simulink model "thermostate"  (R2026a)
settings: Solver=VariableStepAuto  StopTime=1800
undefined symbols (not defined in the file): cp, eta, m_water, P_heater, T_ambient, T_high, T_initial, T_low, t_stop, UA
settings Model: Creator=a  LastModifiedBy=a

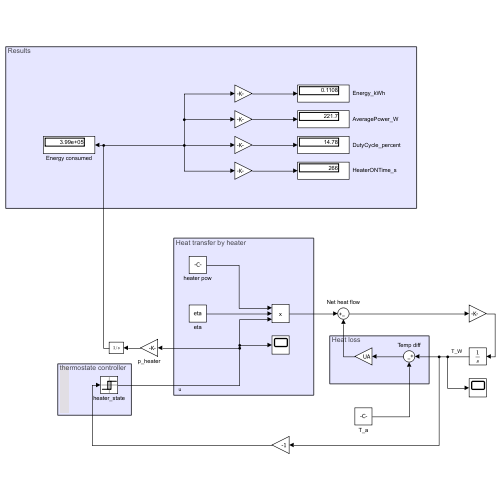
[thumbnail: Simulink's stored preview of the top-level diagram]
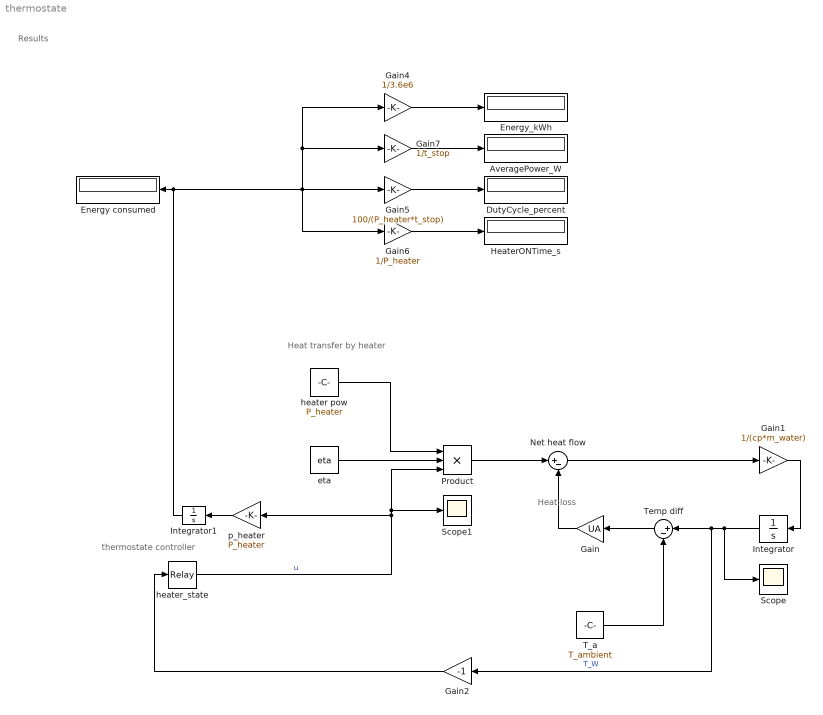
== system thermostate ==
  note: Results
  note: thermostate controller
  note: Heat loss
  note: Heat transfer by heater
  AveragePower_W : Display
  DutyCycle_percent : Display
  Energy consumed : Display
  Energy_kWh : Display
  Gain : Gain  Gain=UA
  Gain1 : Gain  Gain=1/(cp*m_water)
  Gain2 : Gain  Gain=-1
  Gain4 : Gain  Gain=1/3.6e6
  Gain5 : Gain  Gain=100/(P_heater*t_stop)
  Gain6 : Gain  Gain=1/P_heater
  Gain7 : Gain  Gain=1/t_stop
  HeaterONTime_s : Display
  Integrator : Integrator  InitialCondition=T_initial
  Integrator1 : Integrator
  Net heat flow : Sum  Inputs=|+-
  Product : Product  Inputs=3
  Scope : Scope
      settings: ActiveDisplayYMinimum=21.874999999999964  ActiveDisplayYMaximum=53.125000000000334
  Scope1 : Scope
      settings: ActiveDisplayYMinimum=-0.12499999999999997  ActiveDisplayYMaximum=1.125
  T_a : Constant  Value=T_ambient
  Temp diff : Sum  Inputs=|+-
  eta : Constant  Value=eta
  heater pow : Constant  Value=P_heater
  heater_state : Relay  OnSwitchValue=-T_low  OffSwitchValue=-T_high
  p_heater : Gain  Gain=P_heater
  wires:
  heater pow/1 -> Product/1
  eta/1 -> Product/2
  heater_state/1 -> Scope1/1, Product/3, p_heater/1  "u"
  Product/1 -> Net heat flow/1
  Gain/1 -> Net heat flow/2
  Integrator/1 -> Scope/1, Gain2/1, Temp diff/1  "T_W"
  T_a/1 -> Temp diff/2
  Gain1/1 -> Integrator/1
  Net heat flow/1 -> Gain1/1
  Temp diff/1 -> Gain/1
  Gain2/1 -> heater_state/1
  p_heater/1 -> Integrator1/1
  Integrator1/1 -> Gain4/1, Gain7/1, Gain6/1, Gain5/1, Energy consumed/1
  Gain4/1 -> Energy_kWh/1
  Gain7/1 -> AveragePower_W/1
  Gain5/1 -> DutyCycle_percent/1
  Gain6/1 -> HeaterONTime_s/1
